simulink model "ASM_Traffic"  (R2026a)
settings: Solver=ode1  StartTime=SIM.tstart.v  StopTime=SIM.tend.v  FixedStep=SIM.StepSize.v
PostLoadFcn:
  | if any(exist('dsrtsu_mdlpostloadfcn', 'file') ~= 0), dsrtsu_mdlpostloadfcn('Execute', bdroot); end
  | try, asm_mdl_postloadfcn(bdroot, 'UpdateModel', 3600); catch, disp(lasterr); end,
InitFcn:
  | , if any(exist('rtifpga_mdlclblib', 'file') ~= 0), rtifpga_mdlclblib('Init', bdroot); end,
  | , if any(exist('dsmpb_private', 'file') ~= 0), dsmpb_private('dsmpb_mdlclblib', 'Init', bdroot); end,
model workspace (MAT data in the model file):
  asmReferencePath = [0 0.01 0.02 0.03 0.04 0.05 0.06 0.07 0.08 0.09 0.1 0.11 ... (350007 elements, 50001x7)]
  roadBounds : Simulink.Parameter (value not decoded)
  safetyAxes : Simulink.Parameter (value not decoded)
undefined symbols (not defined in the file): _to_, a0b2, ASM_BrakeHydraulics_DemoSystems, ASM_VehicleDynamics_DemoSystems, b98103fe8ad365046cd0, BrakeCircuit, controllerConfig, CPT, Crankshaft, DiscIntNeverNeededParam, dsmsi, FinalDriveAssembly, MDL, ModeSignals, mu, Pos_BrakePedal_Maneuver, rad, RefSignals, roadFamilyData, roadFamilyId, s_to_rpm, SIM, SoftECU, Suspension, Tire, Transmission
libraries: ASM_Traffic_lib x135, simulink x98, ASM_Utils_lib x77, ASM_VehicleDynamics_lib x70, ASM_Environment_lib x22, dsmpblib x20, dsmsilib x15, MDLD_Utils_lib x10, ASM_BrakeHydraulics_lib x3, sl_discontinuities x2
(part 51 of 65)

== system ASM_Traffic/Environment/Sensors/UserInterface/DISP_Plant/Object_Sensor_2D/GetSensorData_2DSensor_6 ==
  TrafficBus : Inport
  Bus Selector1 : BusSelector  OutputSignals=SensorStatus.Flag_Object_In_Scope[0Out|1In],SensorStatus.Flag_Sensor_Apex_In_Object[0Out|1In],SensorOutput.Angle_Hor_Rel[deg],SensorOutput.Object_ID[],SensorOutput.Object_Type[],SensorOutput.Distance[m],SensorOutput.v_Rel[m|s],SensorOutput.a_Rel[m|s2],SensorOutput.Height_Min[m],SensorOutput.Height_Max[m]
  Flag_Object_In_Scope[0Out|1In] : Outport  VectorParamsAs1DForOutWhenUnconnected=off
  Flag_Sensor_Apex_In_Object[0Out|1In] : Outport  Port=2  VectorParamsAs1DForOutWhenUnconnected=off
  Angle_Hor_Rel[deg] : Outport  Port=3  VectorParamsAs1DForOutWhenUnconnected=off
  Object_ID[] : Outport  Port=4  VectorParamsAs1DForOutWhenUnconnected=off
  Object_Type[] : Outport  Port=5  VectorParamsAs1DForOutWhenUnconnected=off
  Distance[m] : Outport  Port=6  VectorParamsAs1DForOutWhenUnconnected=off
  v_Rel[m|s] : Outport  Port=7  VectorParamsAs1DForOutWhenUnconnected=off
  a_Rel[m|s2] : Outport  Port=8  VectorParamsAs1DForOutWhenUnconnected=off
  Height_Min[m] : Outport  Port=9  VectorParamsAs1DForOutWhenUnconnected=off
  Height_Max[m] : Outport  Port=10  VectorParamsAs1DForOutWhenUnconnected=off
  wires:
  TrafficBus/1 -> Bus Selector1/1
  Bus Selector1/3 -> Angle_Hor_Rel[deg]/1  "<Angle_Hor_Rel[deg]>"
  Bus Selector1/4 -> Object_ID[]/1  "<Object_ID[]>"
  Bus Selector1/5 -> Object_Type[]/1  "<Object_Type[]>"
  Bus Selector1/6 -> Distance[m]/1  "<Distance[m]>"
  Bus Selector1/7 -> v_Rel[m|s]/1  "<v_Rel[m|s]>"
  Bus Selector1/8 -> a_Rel[m|s2]/1  "<a_Rel[m|s2]>"
  Bus Selector1/9 -> Height_Min[m]/1  "<Height_Min[m]>"
  Bus Selector1/10 -> Height_Max[m]/1  "<Height_Max[m]>"
  Bus Selector1/1 -> Flag_Object_In_Scope[0Out|1In]/1  "<Flag_Object_In_Scope[0Out|1In]>"
  Bus Selector1/2 -> Flag_Sensor_Apex_In_Object[0Out|1In]/1  "<Flag_Sensor_Apex_In_Object[0Out|1In]>"

== system ASM_Traffic/Environment/Sensors/UserInterface/DISP_Plant/Object_Sensor_2D/GetSensorData_2DSensor_7 ==
  TrafficBus : Inport
  Bus Selector1 : BusSelector  OutputSignals=SensorStatus.Flag_Object_In_Scope[0Out|1In],SensorStatus.Flag_Sensor_Apex_In_Object[0Out|1In],SensorOutput.Angle_Hor_Rel[deg],SensorOutput.Object_ID[],SensorOutput.Object_Type[],SensorOutput.Distance[m],SensorOutput.v_Rel[m|s],SensorOutput.a_Rel[m|s2],SensorOutput.Height_Min[m],SensorOutput.Height_Max[m]
  Flag_Object_In_Scope[0Out|1In] : Outport  VectorParamsAs1DForOutWhenUnconnected=off
  Flag_Sensor_Apex_In_Object[0Out|1In] : Outport  Port=2  VectorParamsAs1DForOutWhenUnconnected=off
  Angle_Hor_Rel[deg] : Outport  Port=3  VectorParamsAs1DForOutWhenUnconnected=off
  Object_ID[] : Outport  Port=4  VectorParamsAs1DForOutWhenUnconnected=off
  Object_Type[] : Outport  Port=5  VectorParamsAs1DForOutWhenUnconnected=off
  Distance[m] : Outport  Port=6  VectorParamsAs1DForOutWhenUnconnected=off
  v_Rel[m|s] : Outport  Port=7  VectorParamsAs1DForOutWhenUnconnected=off
  a_Rel[m|s2] : Outport  Port=8  VectorParamsAs1DForOutWhenUnconnected=off
  Height_Min[m] : Outport  Port=9  VectorParamsAs1DForOutWhenUnconnected=off
  Height_Max[m] : Outport  Port=10  VectorParamsAs1DForOutWhenUnconnected=off
  wires:
  Bus Selector1/2 -> Flag_Sensor_Apex_In_Object[0Out|1In]/1  "<Flag_Sensor_Apex_In_Object[0Out|1In]>"
  Bus Selector1/1 -> Flag_Object_In_Scope[0Out|1In]/1  "<Flag_Object_In_Scope[0Out|1In]>"
  Bus Selector1/10 -> Height_Max[m]/1  "<Height_Max[m]>"
  Bus Selector1/9 -> Height_Min[m]/1  "<Height_Min[m]>"
  Bus Selector1/8 -> a_Rel[m|s2]/1  "<a_Rel[m|s2]>"
  Bus Selector1/7 -> v_Rel[m|s]/1  "<v_Rel[m|s]>"
  Bus Selector1/6 -> Distance[m]/1  "<Distance[m]>"
  Bus Selector1/5 -> Object_Type[]/1  "<Object_Type[]>"
  Bus Selector1/4 -> Object_ID[]/1  "<Object_ID[]>"
  Bus Selector1/3 -> Angle_Hor_Rel[deg]/1  "<Angle_Hor_Rel[deg]>"
  TrafficBus/1 -> Bus Selector1/1

== system ASM_Traffic/Environment/Sensors/UserInterface/DISP_Plant/Object_Sensor_2D/Height_Max[m] ==
  In1 : Inport
  Out1 : Outport  VectorParamsAs1DForOutWhenUnconnected=off
  wires:
  In1/1 -> Out1/1

== system ASM_Traffic/Environment/Sensors/UserInterface/DISP_Plant/Object_Sensor_2D/Height_Max[m]1 ==
  In1 : Inport
  Out1 : Outport  VectorParamsAs1DForOutWhenUnconnected=off
  wires:
  In1/1 -> Out1/1

== system ASM_Traffic/Environment/Sensors/UserInterface/DISP_Plant/Object_Sensor_2D/Height_Max[m]2 ==
  In1 : Inport
  Out1 : Outport  VectorParamsAs1DForOutWhenUnconnected=off
  wires:
  In1/1 -> Out1/1

== system ASM_Traffic/Environment/Sensors/UserInterface/DISP_Plant/Object_Sensor_2D/Height_Max[m]3 ==
  In1 : Inport
  Out1 : Outport  VectorParamsAs1DForOutWhenUnconnected=off
  wires:
  In1/1 -> Out1/1

== system ASM_Traffic/Environment/Sensors/UserInterface/DISP_Plant/Object_Sensor_2D/Height_Max[m]4 ==
  In1 : Inport
  Out1 : Outport  VectorParamsAs1DForOutWhenUnconnected=off
  wires:
  In1/1 -> Out1/1

== system ASM_Traffic/Environment/Sensors/UserInterface/DISP_Plant/Object_Sensor_2D/Height_Max[m]5 ==
  In1 : Inport
  Out1 : Outport  VectorParamsAs1DForOutWhenUnconnected=off
  wires:
  In1/1 -> Out1/1

== system ASM_Traffic/Environment/Sensors/UserInterface/DISP_Plant/Object_Sensor_2D/Height_Max[m]6 ==
  In1 : Inport
  Out1 : Outport  VectorParamsAs1DForOutWhenUnconnected=off
  wires:
  In1/1 -> Out1/1

== system ASM_Traffic/Environment/Sensors/UserInterface/DISP_Plant/Object_Sensor_2D/Height_Min[m] ==
  In1 : Inport
  Out1 : Outport  VectorParamsAs1DForOutWhenUnconnected=off
  wires:
  In1/1 -> Out1/1

== system ASM_Traffic/Environment/Sensors/UserInterface/DISP_Plant/Object_Sensor_2D/Height_Min[m]1 ==
  In1 : Inport
  Out1 : Outport  VectorParamsAs1DForOutWhenUnconnected=off
  wires:
  In1/1 -> Out1/1

== system ASM_Traffic/Environment/Sensors/UserInterface/DISP_Plant/Object_Sensor_2D/Height_Min[m]2 ==
  In1 : Inport
  Out1 : Outport  VectorParamsAs1DForOutWhenUnconnected=off
  wires:
  In1/1 -> Out1/1

== system ASM_Traffic/Environment/Sensors/UserInterface/DISP_Plant/Object_Sensor_2D/Height_Min[m]3 ==
  In1 : Inport
  Out1 : Outport  VectorParamsAs1DForOutWhenUnconnected=off
  wires:
  In1/1 -> Out1/1

== system ASM_Traffic/Environment/Sensors/UserInterface/DISP_Plant/Object_Sensor_2D/Height_Min[m]4 ==
  In1 : Inport
  Out1 : Outport  VectorParamsAs1DForOutWhenUnconnected=off
  wires:
  In1/1 -> Out1/1

== system ASM_Traffic/Environment/Sensors/UserInterface/DISP_Plant/Object_Sensor_2D/Height_Min[m]5 ==
  In1 : Inport
  Out1 : Outport  VectorParamsAs1DForOutWhenUnconnected=off
  wires:
  In1/1 -> Out1/1

== system ASM_Traffic/Environment/Sensors/UserInterface/DISP_Plant/Object_Sensor_2D/Height_Min[m]6 ==
  In1 : Inport
  Out1 : Outport  VectorParamsAs1DForOutWhenUnconnected=off
  wires:
  In1/1 -> Out1/1

== system ASM_Traffic/Environment/Sensors/UserInterface/DISP_Plant/Object_Sensor_2D/IdxSelect_2DSensor ==
  Sensor_1 : Inport
  Sensor_2 : Inport  Port=2
  Sensor_3 : Inport  Port=3
  Sensor_4 : Inport  Port=4
  Sensor_5 : Inport  Port=5
  Sensor_6 : Inport  Port=6
  Sensor_7 : Inport  Port=7
  Bus Selector2 : BusSelector  OutputSignals=SensorStatus.Flag_Object_In_Scope[0Out|1In],SensorStatus.Flag_Sensor_Apex_In_Object[0Out|1In],SensorOutput.Angle_Hor_Rel[deg],SensorOutput.Object_ID[],SensorOutput.Object_Type[],SensorOutput.Distance[m],SensorOutput.v_Rel[m|s],SensorOutput.a_Rel[m|s2],SensorOutput.Height_Min[m],SensorOutput.Height_Max[m]
  Const_Scopezon_El_Idx_1[1_60] : Constant
  Const_Scopezon_El_Idx_2[1_60] : Constant  Value=2
  Const_Scopezon_El_Idx_3[1_60] : Constant  Value=3
  Const_Scopezon_El_Idx_4[1_60] : Constant  Value=4
  Const_Scopezon_El_Idx_5[1_60] : Constant  Value=5
  Multiport Switch : MultiPortSwitch  Inputs=7  SaturateOnIntegerOverflow=off  InputSameDT=off
  Scopezone_Element_Data_Selection1 : Subsystem
  Scopezone_Element_Data_Selection2 : Subsystem
  Scopezone_Element_Data_Selection3 : Subsystem
  Scopezone_Element_Data_Selection4 : Subsystem
  Scopezone_Element_Data_Selection5 : Subsystem
  Sw_Sensor_Selector[] : Constant
  wires:
  Const_Scopezon_El_Idx_5[1_60]/1 -> Scopezone_Element_Data_Selection5/1(Scopezone_El_Idx[1_60])
  Const_Scopezon_El_Idx_4[1_60]/1 -> Scopezone_Element_Data_Selection4/1(Scopezone_El_Idx[1_60])
  Const_Scopezon_El_Idx_3[1_60]/1 -> Scopezone_Element_Data_Selection3/1(Scopezone_El_Idx[1_60])
  Const_Scopezon_El_Idx_2[1_60]/1 -> Scopezone_Element_Data_Selection2/1(Scopezone_El_Idx[1_60])
  Const_Scopezon_El_Idx_1[1_60]/1 -> Scopezone_Element_Data_Selection1/1(Scopezone_El_Idx[1_60])
  Multiport Switch/1 -> Bus Selector2/1
  Bus Selector2/3 -> Scopezone_Element_Data_Selection1/4(Angle_Hor_Rel[deg]), Scopezone_Element_Data_Selection4/4(Angle_Hor_Rel[deg]), Scopezone_Element_Data_Selection5/4(Angle_Hor_Rel[deg]), Scopezone_Element_Data_Selection3/4(Angle_Hor_Rel[deg]), Scopezone_Element_Data_Selection2/4(Angle_Hor_Rel[deg])  "<Angle_Hor_Rel[deg]>"
  Bus Selector2/4 -> Scopezone_Element_Data_Selection4/5(Object_ID[]), Scopezone_Element_Data_Selection5/5(Object_ID[]), Scopezone_Element_Data_Selection3/5(Object_ID[]), Scopezone_Element_Data_Selection2/5(Object_ID[]), Scopezone_Element_Data_Selection1/5(Object_ID[])  "<Object_ID[]>"
  Bus Selector2/5 -> Scopezone_Element_Data_Selection3/6(Object_Type[]), Scopezone_Element_Data_Selection4/6(Object_Type[]), Scopezone_Element_Data_Selection5/6(Object_Type[]), Scopezone_Element_Data_Selection2/6(Object_Type[]), Scopezone_Element_Data_Selection1/6(Object_Type[])  "<Object_Type[]>"
  Bus Selector2/6 -> Scopezone_Element_Data_Selection4/7(Distance[m]), Scopezone_Element_Data_Selection5/7(Distance[m]), Scopezone_Element_Data_Selection3/7(Distance[m]), Scopezone_Element_Data_Selection2/7(Distance[m]), Scopezone_Element_Data_Selection1/7(Distance[m])  "<Distance[m]>"
  Bus Selector2/7 -> Scopezone_Element_Data_Selection4/8(v_Rel[m|s]), Scopezone_Element_Data_Selection5/8(v_Rel[m|s]), Scopezone_Element_Data_Selection3/8(v_Rel[m|s]), Scopezone_Element_Data_Selection2/8(v_Rel[m|s]), Scopezone_Element_Data_Selection1/8(v_Rel[m|s])  "<v_Rel[m|s]>"
  Bus Selector2/8 -> Scopezone_Element_Data_Selection4/9(a_Rel[m|s2]), Scopezone_Element_Data_Selection5/9(a_Rel[m|s2]), Scopezone_Element_Data_Selection3/9(a_Rel[m|s2]), Scopezone_Element_Data_Selection2/9(a_Rel[m|s2]), Scopezone_Element_Data_Selection1/9(a_Rel[m|s2])  "<a_Rel[m|s2]>"
  Bus Selector2/9 -> Scopezone_Element_Data_Selection4/10(Height_Min[m]), Scopezone_Element_Data_Selection5/10(Height_Min[m]), Scopezone_Element_Data_Selection3/10(Height_Min[m]), Scopezone_Element_Data_Selection2/10(Height_Min[m]), Scopezone_Element_Data_Selection1/10(Height_Min[m])  "<Height_Min[m]>"
  Bus Selector2/10 -> Scopezone_Element_Data_Selection4/11(Height_Max[m]), Scopezone_Element_Data_Selection5/11(Height_Max[m]), Scopezone_Element_Data_Selection3/11(Height_Max[m]), Scopezone_Element_Data_Selection2/11(Height_Max[m]), Scopezone_Element_Data_Selection1/11(Height_Max[m])  "<Height_Max[m]>"
  Bus Selector2/1 -> Scopezone_Element_Data_Selection1/2(Flag_Object_In_Scope[0Out|1In]), Scopezone_Element_Data_Selection4/2(Flag_Object_In_Scope[0Out|1In]), Scopezone_Element_Data_Selection5/2(Flag_Object_In_Scope[0Out|1In]), Scopezone_Element_Data_Selection3/2(Flag_Object_In_Scope[0Out|1In]), Scopezone_Element_Data_Selection2/2(Flag_Object_In_Scope[0Out|1In])  "<Flag_Object_In_Scope[0Out|1In]>"
  Bus Selector2/2 -> Scopezone_Element_Data_Selection1/3(Flag_Sensor_Apex_In_Object[0Out|1In]), Scopezone_Element_Data_Selection4/3(Flag_Sensor_Apex_In_Object[0Out|1In]), Scopezone_Element_Data_Selection5/3(Flag_Sensor_Apex_In_Object[0Out|1In]), Scopezone_Element_Data_Selection3/3(Flag_Sensor_Apex_In_Object[0Out|1In]), Scopezone_Element_Data_Selection2/3(Flag_Sensor_Apex_In_Object[0Out|1In])  "<Flag_Sensor_Apex_In_Object[0Out|1In]>"
  Sensor_7/1 -> Multiport Switch/8
  Sensor_6/1 -> Multiport Switch/7
  Sensor_5/1 -> Multiport Switch/6
  Sensor_4/1 -> Multiport Switch/5
  Sw_Sensor_Selector[]/1 -> Multiport Switch/1
  Sensor_1/1 -> Multiport Switch/2
  Sensor_2/1 -> Multiport Switch/3
  Sensor_3/1 -> Multiport Switch/4

== system ASM_Traffic/Environment/Sensors/UserInterface/DISP_Plant/Object_Sensor_2D/IndexConflict_Info[] ==
  In1 : Inport
  Out1 : Outport  VectorParamsAs1DForOutWhenUnconnected=off
  wires:
  In1/1 -> Out1/1

== system ASM_Traffic/Environment/Sensors/UserInterface/DISP_Plant/Object_Sensor_2D/InputDataSamplePulse[0|1] ==
  In1 : Inport
  Out1 : Outport  VectorParamsAs1DForOutWhenUnconnected=off
  wires:
  In1/1 -> Out1/1

== system ASM_Traffic/Environment/Sensors/UserInterface/DISP_Plant/Object_Sensor_2D/ObjectSensor2D_Data_Valid[0|1] ==
  In1 : Inport
  Out1 : Outport  VectorParamsAs1DForOutWhenUnconnected=off
  wires:
  In1/1 -> Out1/1

== system ASM_Traffic/Environment/Sensors/UserInterface/DISP_Plant/Object_Sensor_2D/ObjectSensor2D_Sfcn_State[] ==
  In1 : Inport
  Out1 : Outport  VectorParamsAs1DForOutWhenUnconnected=off
  wires:
  In1/1 -> Out1/1

== system ASM_Traffic/Environment/Sensors/UserInterface/DISP_Plant/Object_Sensor_2D/Object_ID[] ==
  In1 : Inport
  Out1 : Outport  VectorParamsAs1DForOutWhenUnconnected=off
  wires:
  In1/1 -> Out1/1

== system ASM_Traffic/Environment/Sensors/UserInterface/DISP_Plant/Object_Sensor_2D/Object_ID[]1 ==
  In1 : Inport
  Out1 : Outport  VectorParamsAs1DForOutWhenUnconnected=off
  wires:
  In1/1 -> Out1/1

== system ASM_Traffic/Environment/Sensors/UserInterface/DISP_Plant/Object_Sensor_2D/Object_ID[]2 ==
  In1 : Inport
  Out1 : Outport  VectorParamsAs1DForOutWhenUnconnected=off
  wires:
  In1/1 -> Out1/1

== system ASM_Traffic/Environment/Sensors/UserInterface/DISP_Plant/Object_Sensor_2D/Object_ID[]3 ==
  In1 : Inport
  Out1 : Outport  VectorParamsAs1DForOutWhenUnconnected=off
  wires:
  In1/1 -> Out1/1

== system ASM_Traffic/Environment/Sensors/UserInterface/DISP_Plant/Object_Sensor_2D/Object_ID[]4 ==
  In1 : Inport
  Out1 : Outport  VectorParamsAs1DForOutWhenUnconnected=off
  wires:
  In1/1 -> Out1/1

== system ASM_Traffic/Environment/Sensors/UserInterface/DISP_Plant/Object_Sensor_2D/Object_ID[]5 ==
  In1 : Inport
  Out1 : Outport  VectorParamsAs1DForOutWhenUnconnected=off
  wires:
  In1/1 -> Out1/1

== system ASM_Traffic/Environment/Sensors/UserInterface/DISP_Plant/Object_Sensor_2D/Object_ID[]6 ==
  In1 : Inport
  Out1 : Outport  VectorParamsAs1DForOutWhenUnconnected=off
  wires:
  In1/1 -> Out1/1

== system ASM_Traffic/Environment/Sensors/UserInterface/DISP_Plant/Object_Sensor_2D/Object_Sensor_2D_VisualizationData ==
  TrafficBus : Inport
  Bus Selector9 : BusSelector  OutputSignals=Object_Sensor_2D.Sensor_1_Front,Object_Sensor_2D.Sensor_2_Front_Left,Object_Sensor_2D.Sensor_3_Left,Object_Sensor_2D.Sensor_4_Rear_Left,Object_Sensor_2D.Sensor_5_Front_Right,Object_Sensor_2D.Sensor_6_Right,Object_Sensor_2D.Sensor_7_Rear_Right
  Sensor_1_Front_Long : Subsystem
  Sensor_2_Front_Left : Subsystem
  Sensor_3_Left : Subsystem
  Sensor_4_Rear_Left : Subsystem
  Sensor_5_Front_Right : Subsystem
  Sensor_6_Right : Subsystem
  Sensor_7_Rear_Right : Subsystem
  wires:
  Bus Selector9/1 -> Sensor_1_Front_Long/1(Sensor)  "<Sensor_1_Front>"
  TrafficBus/1 -> Bus Selector9/1
  Bus Selector9/2 -> Sensor_2_Front_Left/1(Sensor)  "<Sensor_2_Front_Left>"
  Bus Selector9/3 -> Sensor_3_Left/1(Sensor)  "<Sensor_3_Left>"
  Bus Selector9/4 -> Sensor_4_Rear_Left/1(Sensor)  "<Sensor_4_Rear_Left>"
  Bus Selector9/5 -> Sensor_5_Front_Right/1(Sensor)  "<Sensor_5_Front_Right>"
  Bus Selector9/6 -> Sensor_6_Right/1(Sensor)  "<Sensor_6_Right>"
  Bus Selector9/7 -> Sensor_7_Rear_Right/1(Sensor)  "<Sensor_7_Rear_Right>"

== system ASM_Traffic/Environment/Sensors/UserInterface/DISP_Plant/Object_Sensor_2D/Object_Type[] ==
  In1 : Inport
  Out1 : Outport  VectorParamsAs1DForOutWhenUnconnected=off
  wires:
  In1/1 -> Out1/1

== system ASM_Traffic/Environment/Sensors/UserInterface/DISP_Plant/Object_Sensor_2D/Object_Type[]1 ==
  In1 : Inport
  Out1 : Outport  VectorParamsAs1DForOutWhenUnconnected=off
  wires:
  In1/1 -> Out1/1

== system ASM_Traffic/Environment/Sensors/UserInterface/DISP_Plant/Object_Sensor_2D/Object_Type[]2 ==
  In1 : Inport
  Out1 : Outport  VectorParamsAs1DForOutWhenUnconnected=off
  wires:
  In1/1 -> Out1/1

== system ASM_Traffic/Environment/Sensors/UserInterface/DISP_Plant/Object_Sensor_2D/Object_Type[]3 ==
  In1 : Inport
  Out1 : Outport  VectorParamsAs1DForOutWhenUnconnected=off
  wires:
  In1/1 -> Out1/1

== system ASM_Traffic/Environment/Sensors/UserInterface/DISP_Plant/Object_Sensor_2D/Object_Type[]4 ==
  In1 : Inport
  Out1 : Outport  VectorParamsAs1DForOutWhenUnconnected=off
  wires:
  In1/1 -> Out1/1

== system ASM_Traffic/Environment/Sensors/UserInterface/DISP_Plant/Object_Sensor_2D/Object_Type[]5 ==
  In1 : Inport
  Out1 : Outport  VectorParamsAs1DForOutWhenUnconnected=off
  wires:
  In1/1 -> Out1/1

== system ASM_Traffic/Environment/Sensors/UserInterface/DISP_Plant/Object_Sensor_2D/Object_Type[]6 ==
  In1 : Inport
  Out1 : Outport  VectorParamsAs1DForOutWhenUnconnected=off
  wires:
  In1/1 -> Out1/1

== system ASM_Traffic/Environment/Sensors/UserInterface/DISP_Plant/Object_Sensor_2D/SensorEnable[0Off|1On] ==
  In1 : Inport
  Out1 : Outport  VectorParamsAs1DForOutWhenUnconnected=off
  wires:
  In1/1 -> Out1/1

== system ASM_Traffic/Environment/Sensors/UserInterface/DISP_Plant/Object_Sensor_2D/SensorIdx_Selected[] ==
  In1 : Inport
  Out1 : Outport  VectorParamsAs1DForOutWhenUnconnected=off
  wires:
  In1/1 -> Out1/1

== system ASM_Traffic/Environment/Sensors/UserInterface/DISP_Plant/Object_Sensor_2D/SensorSelection_Data[0|1] ==
  In1 : Inport
  Out1 : Outport  VectorParamsAs1DForOutWhenUnconnected=off
  wires:
  In1/1 -> Out1/1

== system ASM_Traffic/Environment/Sensors/UserInterface/DISP_Plant/Object_Sensor_2D/a_Rel[m|s2] ==
  In1 : Inport
  Out1 : Outport  VectorParamsAs1DForOutWhenUnconnected=off
  wires:
  In1/1 -> Out1/1

== system ASM_Traffic/Environment/Sensors/UserInterface/DISP_Plant/Object_Sensor_2D/a_Rel[m|s2]1 ==
  In1 : Inport
  Out1 : Outport  VectorParamsAs1DForOutWhenUnconnected=off
  wires:
  In1/1 -> Out1/1

== system ASM_Traffic/Environment/Sensors/UserInterface/DISP_Plant/Object_Sensor_2D/a_Rel[m|s2]2 ==
  In1 : Inport
  Out1 : Outport  VectorParamsAs1DForOutWhenUnconnected=off
  wires:
  In1/1 -> Out1/1

== system ASM_Traffic/Environment/Sensors/UserInterface/DISP_Plant/Object_Sensor_2D/a_Rel[m|s2]3 ==
  In1 : Inport
  Out1 : Outport  VectorParamsAs1DForOutWhenUnconnected=off
  wires:
  In1/1 -> Out1/1

== system ASM_Traffic/Environment/Sensors/UserInterface/DISP_Plant/Object_Sensor_2D/a_Rel[m|s2]4 ==
  In1 : Inport
  Out1 : Outport  VectorParamsAs1DForOutWhenUnconnected=off
  wires:
  In1/1 -> Out1/1

== system ASM_Traffic/Environment/Sensors/UserInterface/DISP_Plant/Object_Sensor_2D/a_Rel[m|s2]5 ==
  In1 : Inport
  Out1 : Outport  VectorParamsAs1DForOutWhenUnconnected=off
  wires:
  In1/1 -> Out1/1

== system ASM_Traffic/Environment/Sensors/UserInterface/DISP_Plant/Object_Sensor_2D/a_Rel[m|s2]6 ==
  In1 : Inport
  Out1 : Outport  VectorParamsAs1DForOutWhenUnconnected=off
  wires:
  In1/1 -> Out1/1

== system ASM_Traffic/Environment/Sensors/UserInterface/DISP_Plant/Object_Sensor_2D/v_Rel[m|s] ==
  In1 : Inport
  Out1 : Outport  VectorParamsAs1DForOutWhenUnconnected=off
  wires:
  In1/1 -> Out1/1

== system ASM_Traffic/Environment/Sensors/UserInterface/DISP_Plant/Object_Sensor_2D/v_Rel[m|s]1 ==
  In1 : Inport
  Out1 : Outport  VectorParamsAs1DForOutWhenUnconnected=off
  wires:
  In1/1 -> Out1/1

== system ASM_Traffic/Environment/Sensors/UserInterface/DISP_Plant/Object_Sensor_2D/v_Rel[m|s]2 ==
  In1 : Inport
  Out1 : Outport  VectorParamsAs1DForOutWhenUnconnected=off
  wires:
  In1/1 -> Out1/1

== system ASM_Traffic/Environment/Sensors/UserInterface/DISP_Plant/Object_Sensor_2D/v_Rel[m|s]3 ==
  In1 : Inport
  Out1 : Outport  VectorParamsAs1DForOutWhenUnconnected=off
  wires:
  In1/1 -> Out1/1

== system ASM_Traffic/Environment/Sensors/UserInterface/DISP_Plant/Object_Sensor_2D/v_Rel[m|s]4 ==
  In1 : Inport
  Out1 : Outport  VectorParamsAs1DForOutWhenUnconnected=off
  wires:
  In1/1 -> Out1/1

== system ASM_Traffic/Environment/Sensors/UserInterface/DISP_Plant/Object_Sensor_2D/v_Rel[m|s]5 ==
  In1 : Inport
  Out1 : Outport  VectorParamsAs1DForOutWhenUnconnected=off
  wires:
  In1/1 -> Out1/1

== system ASM_Traffic/Environment/Sensors/UserInterface/DISP_Plant/Object_Sensor_2D/v_Rel[m|s]6 ==
  In1 : Inport
  Out1 : Outport  VectorParamsAs1DForOutWhenUnconnected=off
  wires:
  In1/1 -> Out1/1

== system ASM_Traffic/Environment/Sensors/UserInterface/DISP_Plant/Object_Sensor_3D/Angle_Hor_Object[deg] ==
  In1 : Inport
  Out1 : Outport  VectorParamsAs1DForOutWhenUnconnected=off
  wires:
  In1/1 -> Out1/1

== system ASM_Traffic/Environment/Sensors/UserInterface/DISP_Plant/Object_Sensor_3D/Angle_Hor_Object[deg]1 ==
  In1 : Inport
  Out1 : Outport  VectorParamsAs1DForOutWhenUnconnected=off
  wires:
  In1/1 -> Out1/1

== system ASM_Traffic/Environment/Sensors/UserInterface/DISP_Plant/Object_Sensor_3D/Angle_Hor_Object[deg]2 ==
  In1 : Inport
  Out1 : Outport  VectorParamsAs1DForOutWhenUnconnected=off
  wires:
  In1/1 -> Out1/1

== system ASM_Traffic/Environment/Sensors/UserInterface/DISP_Plant/Object_Sensor_3D/Angle_Ver_Object[deg] ==
  In1 : Inport
  Out1 : Outport  VectorParamsAs1DForOutWhenUnconnected=off
  wires:
  In1/1 -> Out1/1

== system ASM_Traffic/Environment/Sensors/UserInterface/DISP_Plant/Object_Sensor_3D/Angle_Ver_Object[deg]1 ==
  In1 : Inport
  Out1 : Outport  VectorParamsAs1DForOutWhenUnconnected=off
  wires:
  In1/1 -> Out1/1

== system ASM_Traffic/Environment/Sensors/UserInterface/DISP_Plant/Object_Sensor_3D/Angle_Ver_Object[deg]2 ==
  In1 : Inport
  Out1 : Outport  VectorParamsAs1DForOutWhenUnconnected=off
  wires:
  In1/1 -> Out1/1

== system ASM_Traffic/Environment/Sensors/UserInterface/DISP_Plant/Object_Sensor_3D/Conflict_Flag[0|1] ==
  In1 : Inport
  Out1 : Outport  VectorParamsAs1DForOutWhenUnconnected=off
  wires:
  In1/1 -> Out1/1

== system ASM_Traffic/Environment/Sensors/UserInterface/DISP_Plant/Object_Sensor_3D/CycleConflict_Info[] ==
  In1 : Inport
  Out1 : Outport  VectorParamsAs1DForOutWhenUnconnected=off
  wires:
  In1/1 -> Out1/1

== system ASM_Traffic/Environment/Sensors/UserInterface/DISP_Plant/Object_Sensor_3D/DelayPulse_SensorOutput[0|1] ==
  In1 : Inport
  Out1 : Outport  VectorParamsAs1DForOutWhenUnconnected=off
  wires:
  In1/1 -> Out1/1

== system ASM_Traffic/Environment/Sensors/UserInterface/DISP_Plant/Object_Sensor_3D/Dist_Object[m] ==
  In1 : Inport
  Out1 : Outport  VectorParamsAs1DForOutWhenUnconnected=off
  wires:
  In1/1 -> Out1/1

== system ASM_Traffic/Environment/Sensors/UserInterface/DISP_Plant/Object_Sensor_3D/Dist_Object[m]1 ==
  In1 : Inport
  Out1 : Outport  VectorParamsAs1DForOutWhenUnconnected=off
  wires:
  In1/1 -> Out1/1

== system ASM_Traffic/Environment/Sensors/UserInterface/DISP_Plant/Object_Sensor_3D/Dist_Object[m]2 ==
  In1 : Inport
  Out1 : Outport  VectorParamsAs1DForOutWhenUnconnected=off
  wires:
  In1/1 -> Out1/1

== system ASM_Traffic/Environment/Sensors/UserInterface/DISP_Plant/Object_Sensor_3D/Flag_NearestPnt_Occluded[-1|0|1] ==
  In1 : Inport
  Out1 : Outport  VectorParamsAs1DForOutWhenUnconnected=off
  wires:
  In1/1 -> Out1/1

== system ASM_Traffic/Environment/Sensors/UserInterface/DISP_Plant/Object_Sensor_3D/Flag_NearestPnt_Occluded[-1|0|1]1 ==
  In1 : Inport
  Out1 : Outport  VectorParamsAs1DForOutWhenUnconnected=off
  wires:
  In1/1 -> Out1/1

== system ASM_Traffic/Environment/Sensors/UserInterface/DISP_Plant/Object_Sensor_3D/Flag_NearestPnt_Occluded[-1|0|1]2 ==
  In1 : Inport
  Out1 : Outport  VectorParamsAs1DForOutWhenUnconnected=off
  wires:
  In1/1 -> Out1/1

== system ASM_Traffic/Environment/Sensors/UserInterface/DISP_Plant/Object_Sensor_3D/Flag_Object_In_Scope[0Out|1In] ==
  In1 : Inport
  Out1 : Outport  VectorParamsAs1DForOutWhenUnconnected=off
  wires:
  In1/1 -> Out1/1

== system ASM_Traffic/Environment/Sensors/UserInterface/DISP_Plant/Object_Sensor_3D/Flag_Object_In_Scope[0Out|1In]1 ==
  In1 : Inport
  Out1 : Outport  VectorParamsAs1DForOutWhenUnconnected=off
  wires:
  In1/1 -> Out1/1

== system ASM_Traffic/Environment/Sensors/UserInterface/DISP_Plant/Object_Sensor_3D/Flag_Object_In_Scope[0Out|1In]2 ==
  In1 : Inport
  Out1 : Outport  VectorParamsAs1DForOutWhenUnconnected=off
  wires:
  In1/1 -> Out1/1

== system ASM_Traffic/Environment/Sensors/UserInterface/DISP_Plant/Object_Sensor_3D/Flag_Sensor_Apex_In_Object[0Out|1In] ==
  In1 : Inport
  Out1 : Outport  VectorParamsAs1DForOutWhenUnconnected=off
  wires:
  In1/1 -> Out1/1

== system ASM_Traffic/Environment/Sensors/UserInterface/DISP_Plant/Object_Sensor_3D/Flag_Sensor_Apex_In_Object[0Out|1In]1 ==
  In1 : Inport
  Out1 : Outport  VectorParamsAs1DForOutWhenUnconnected=off
  wires:
  In1/1 -> Out1/1

== system ASM_Traffic/Environment/Sensors/UserInterface/DISP_Plant/Object_Sensor_3D/Flag_Sensor_Apex_In_Object[0Out|1In]2 ==
  In1 : Inport
  Out1 : Outport  VectorParamsAs1DForOutWhenUnconnected=off
  wires:
  In1/1 -> Out1/1

== system ASM_Traffic/Environment/Sensors/UserInterface/DISP_Plant/Object_Sensor_3D/GetSensorData_3DSensor_1 ==
  TrafficBus : Inport
  Bus Selector1 : BusSelector  OutputSignals=Info.Flag_Object_In_Scope[0Out|1In],Info.Flag_Sensor_Apex_In_Object[0Out|1In],SensorOutput.Object_Info[-1None|1Fellow|2Static],SensorOutput.Object_ID[],SensorOutput.Object_Type[],SensorOutput.Dist_Object[m],SensorOutput.v_Rel_Object[m|s],SensorOutput.a_Rel_Object[m|s2],SensorOutput.Angle_Hor_Object[deg],SensorOutput.Angle_Ver_Object[deg],SensorOutput.Occlusion_Ratio_Object[-1|0_1],SensorOutput.Flag_NearestPnt_Occluded[-1|0|1]
  Flag_Object_In_Scope[0Out|1In] : Outport  VectorParamsAs1DForOutWhenUnconnected=off
  Flag_Sensor_Apex_In_Object[0Out|1In] : Outport  Port=2  VectorParamsAs1DForOutWhenUnconnected=off
  Object_Info[-1None|1Fellow|2Static] : Outport  Port=3  VectorParamsAs1DForOutWhenUnconnected=off
  Object_ID[] : Outport  Port=4  VectorParamsAs1DForOutWhenUnconnected=off
  Object_Type[] : Outport  Port=5  VectorParamsAs1DForOutWhenUnconnected=off
  Dist_Object[m] : Outport  Port=6  VectorParamsAs1DForOutWhenUnconnected=off
  v_Rel_Object[m|s] : Outport  Port=7  VectorParamsAs1DForOutWhenUnconnected=off
  a_Rel_Object[m|s2] : Outport  Port=8  VectorParamsAs1DForOutWhenUnconnected=off
  Angle_Hor_Object[deg] : Outport  Port=9  VectorParamsAs1DForOutWhenUnconnected=off
  Angle_Ver_Object[deg] : Outport  Port=10  VectorParamsAs1DForOutWhenUnconnected=off
  Occlusion_Ratio_Object[-1|0_1] : Outport  Port=11  VectorParamsAs1DForOutWhenUnconnected=off
  Flag_NearestPnt_Occluded[-1|0|1] : Outport  Port=12  VectorParamsAs1DForOutWhenUnconnected=off
  wires:
  Bus Selector1/12 -> Flag_NearestPnt_Occluded[-1|0|1]/1  "<Flag_NearestPnt_Occluded[-1|0|1]>"
  Bus Selector1/11 -> Occlusion_Ratio_Object[-1|0_1]/1  "<Occlusion_Ratio_Object[-1|0_1]>"
  TrafficBus/1 -> Bus Selector1/1
  Bus Selector1/1 -> Flag_Object_In_Scope[0Out|1In]/1  "<Flag_Object_In_Scope[0Out|1In]>"
  Bus Selector1/2 -> Flag_Sensor_Apex_In_Object[0Out|1In]/1  "<Flag_Sensor_Apex_In_Object[0Out|1In]>"
  Bus Selector1/3 -> Object_Info[-1None|1Fellow|2Static]/1  "<Object_Info[-1None|1Fellow|2Static]>"
  Bus Selector1/4 -> Object_ID[]/1  "<Object_ID[]>"
  Bus Selector1/5 -> Object_Type[]/1  "<Object_Type[]>"
  Bus Selector1/6 -> Dist_Object[m]/1  "<Dist_Object[m]>"
  Bus Selector1/7 -> v_Rel_Object[m|s]/1  "<v_Rel_Object[m|s]>"
  Bus Selector1/8 -> a_Rel_Object[m|s2]/1  "<a_Rel_Object[m|s2]>"
  Bus Selector1/9 -> Angle_Hor_Object[deg]/1  "<Angle_Hor_Object[deg]>"
  Bus Selector1/10 -> Angle_Ver_Object[deg]/1  "<Angle_Ver_Object[deg]>"

== system ASM_Traffic/Environment/Sensors/UserInterface/DISP_Plant/Object_Sensor_3D/GetSensorData_3DSensor_2 ==
  TrafficBus : Inport
  Bus Selector1 : BusSelector  OutputSignals=Info.Flag_Object_In_Scope[0Out|1In],Info.Flag_Sensor_Apex_In_Object[0Out|1In],SensorOutput.Object_Info[-1None|1Fellow|2Static],SensorOutput.Object_ID[],SensorOutput.Object_Type[],SensorOutput.Dist_Object[m],SensorOutput.v_Rel_Object[m|s],SensorOutput.a_Rel_Object[m|s2],SensorOutput.Angle_Hor_Object[deg],SensorOutput.Angle_Ver_Object[deg],SensorOutput.Occlusion_Ratio_Object[-1|0_1],SensorOutput.Flag_NearestPnt_Occluded[-1|0|1]
  Flag_Object_In_Scope[0Out|1In] : Outport  VectorParamsAs1DForOutWhenUnconnected=off
  Flag_Sensor_Apex_In_Object[0Out|1In] : Outport  Port=2  VectorParamsAs1DForOutWhenUnconnected=off
  Object_Info[-1None|1Fellow|2Static] : Outport  Port=3  VectorParamsAs1DForOutWhenUnconnected=off
  Object_ID[] : Outport  Port=4  VectorParamsAs1DForOutWhenUnconnected=off
  Object_Type[] : Outport  Port=5  VectorParamsAs1DForOutWhenUnconnected=off
  Dist_Object[m] : Outport  Port=6  VectorParamsAs1DForOutWhenUnconnected=off
  v_Rel_Object[m|s] : Outport  Port=7  VectorParamsAs1DForOutWhenUnconnected=off
  a_Rel_Object[m|s2] : Outport  Port=8  VectorParamsAs1DForOutWhenUnconnected=off
  Angle_Hor_Object[deg] : Outport  Port=9  VectorParamsAs1DForOutWhenUnconnected=off
  Angle_Ver_Object[deg] : Outport  Port=10  VectorParamsAs1DForOutWhenUnconnected=off
  Occlusion_Ratio_Object[-1|0_1] : Outport  Port=11  VectorParamsAs1DForOutWhenUnconnected=off
  Flag_NearestPnt_Occluded[-1|0|1] : Outport  Port=12  VectorParamsAs1DForOutWhenUnconnected=off
  wires:
  Bus Selector1/12 -> Flag_NearestPnt_Occluded[-1|0|1]/1  "<Flag_NearestPnt_Occluded[-1|0|1]>"
  Bus Selector1/11 -> Occlusion_Ratio_Object[-1|0_1]/1  "<Occlusion_Ratio_Object[-1|0_1]>"
  TrafficBus/1 -> Bus Selector1/1
  Bus Selector1/1 -> Flag_Object_In_Scope[0Out|1In]/1  "<Flag_Object_In_Scope[0Out|1In]>"
  Bus Selector1/2 -> Flag_Sensor_Apex_In_Object[0Out|1In]/1  "<Flag_Sensor_Apex_In_Object[0Out|1In]>"
  Bus Selector1/3 -> Object_Info[-1None|1Fellow|2Static]/1  "<Object_Info[-1None|1Fellow|2Static]>"
  Bus Selector1/4 -> Object_ID[]/1  "<Object_ID[]>"
  Bus Selector1/5 -> Object_Type[]/1  "<Object_Type[]>"
  Bus Selector1/6 -> Dist_Object[m]/1  "<Dist_Object[m]>"
  Bus Selector1/7 -> v_Rel_Object[m|s]/1  "<v_Rel_Object[m|s]>"
  Bus Selector1/8 -> a_Rel_Object[m|s2]/1  "<a_Rel_Object[m|s2]>"
  Bus Selector1/9 -> Angle_Hor_Object[deg]/1  "<Angle_Hor_Object[deg]>"
  Bus Selector1/10 -> Angle_Ver_Object[deg]/1  "<Angle_Ver_Object[deg]>"

== system ASM_Traffic/Environment/Sensors/UserInterface/DISP_Plant/Object_Sensor_3D/GetSensorData_3DSensor_3 ==
  TrafficBus : Inport
  Bus Selector1 : BusSelector  OutputSignals=Info.Flag_Object_In_Scope[0Out|1In],Info.Flag_Sensor_Apex_In_Object[0Out|1In],SensorOutput.Object_Info[-1None|1Fellow|2Static],SensorOutput.Object_ID[],SensorOutput.Object_Type[],SensorOutput.Dist_Object[m],SensorOutput.v_Rel_Object[m|s],SensorOutput.a_Rel_Object[m|s2],SensorOutput.Angle_Hor_Object[deg],SensorOutput.Angle_Ver_Object[deg],SensorOutput.Occlusion_Ratio_Object[-1|0_1],SensorOutput.Flag_NearestPnt_Occluded[-1|0|1]
  Flag_Object_In_Scope[0Out|1In] : Outport  VectorParamsAs1DForOutWhenUnconnected=off
  Flag_Sensor_Apex_In_Object[0Out|1In] : Outport  Port=2  VectorParamsAs1DForOutWhenUnconnected=off
  Object_Info[-1None|1Fellow|2Static] : Outport  Port=3  VectorParamsAs1DForOutWhenUnconnected=off
  Object_ID[] : Outport  Port=4  VectorParamsAs1DForOutWhenUnconnected=off
  Object_Type[] : Outport  Port=5  VectorParamsAs1DForOutWhenUnconnected=off
  Dist_Object[m] : Outport  Port=6  VectorParamsAs1DForOutWhenUnconnected=off
  v_Rel_Object[m|s] : Outport  Port=7  VectorParamsAs1DForOutWhenUnconnected=off
  a_Rel_Object[m|s2] : Outport  Port=8  VectorParamsAs1DForOutWhenUnconnected=off
  Angle_Hor_Object[deg] : Outport  Port=9  VectorParamsAs1DForOutWhenUnconnected=off
  Angle_Ver_Object[deg] : Outport  Port=10  VectorParamsAs1DForOutWhenUnconnected=off
  Occlusion_Ratio_Object[-1|0_1] : Outport  Port=11  VectorParamsAs1DForOutWhenUnconnected=off
  Flag_NearestPnt_Occluded[-1|0|1] : Outport  Port=12  VectorParamsAs1DForOutWhenUnconnected=off
  wires:
  Bus Selector1/12 -> Flag_NearestPnt_Occluded[-1|0|1]/1  "<Flag_NearestPnt_Occluded[-1|0|1]>"
  Bus Selector1/11 -> Occlusion_Ratio_Object[-1|0_1]/1  "<Occlusion_Ratio_Object[-1|0_1]>"
  TrafficBus/1 -> Bus Selector1/1
  Bus Selector1/1 -> Flag_Object_In_Scope[0Out|1In]/1  "<Flag_Object_In_Scope[0Out|1In]>"
  Bus Selector1/2 -> Flag_Sensor_Apex_In_Object[0Out|1In]/1  "<Flag_Sensor_Apex_In_Object[0Out|1In]>"
  Bus Selector1/3 -> Object_Info[-1None|1Fellow|2Static]/1  "<Object_Info[-1None|1Fellow|2Static]>"
  Bus Selector1/4 -> Object_ID[]/1  "<Object_ID[]>"
  Bus Selector1/5 -> Object_Type[]/1  "<Object_Type[]>"
  Bus Selector1/6 -> Dist_Object[m]/1  "<Dist_Object[m]>"
  Bus Selector1/7 -> v_Rel_Object[m|s]/1  "<v_Rel_Object[m|s]>"
  Bus Selector1/8 -> a_Rel_Object[m|s2]/1  "<a_Rel_Object[m|s2]>"
  Bus Selector1/9 -> Angle_Hor_Object[deg]/1  "<Angle_Hor_Object[deg]>"
  Bus Selector1/10 -> Angle_Ver_Object[deg]/1  "<Angle_Ver_Object[deg]>"
